simulink model "P1_secuencia"  (R2025a)
settings: Solver=ode23  StartTime=0.0  StopTime=T_SIM  MaxStep=0.01  RelTol=1e-3
PostLoadFcn:
  | run(fullfile(fileparts(get_param('P1_secuencia', 'FileName')), 'parametros_p1.m'));
InitFcn:
  | run(fullfile(fileparts(get_param('P1_secuencia', 'FileName')), 'parametros_p1.m'));
values from neighbouring files (symbols this model uses):
  CARRERA_13 = 100    [parametros_p1.m]
  CARRERA_45 = 50    [parametros_p1.m]
  DUR_START = 0.3    [parametros_p1.m]
  N_CICLOS = 3    [parametros_p1.m]
  P_CONM = 3    [parametros_p1.m]
  P_MIN_45 = 2    [parametros_p1.m]
  P_RED = 6    [parametros_p1.m]
  T_ESPERA = 1.0    (= 1)    [parametros_p1.m]
  T_NEUM = 5.0    (= 5)    [parametros_p1.m]
  T_START = 0.5    [parametros_p1.m]
  TAU_DESCARGA = 0.05    [parametros_p1.m]
  TAU_LINEA = 0.03    [parametros_p1.m]
  TAU_T1 = RETARDO_T1 / log(P_RED/(P_RED - P_CONM))    [parametros_p1.m]
  TAU_T2 = RETARDO_T2 / log(P_RED/(P_RED - P_CONM))    [parametros_p1.m]
  TOL_SENSOR = 1    [parametros_p1.m]
  V_EXT_13 = 100    [parametros_p1.m]
  V_EXT_45 = 100    [parametros_p1.m]
  V_RET_13 = 100    [parametros_p1.m]
  V_RET_45 = 125    [parametros_p1.m]
libraries: simulink x6
settings Model: Creator=Daan Maldonado  LastModifiedBy=Daan Maldonado

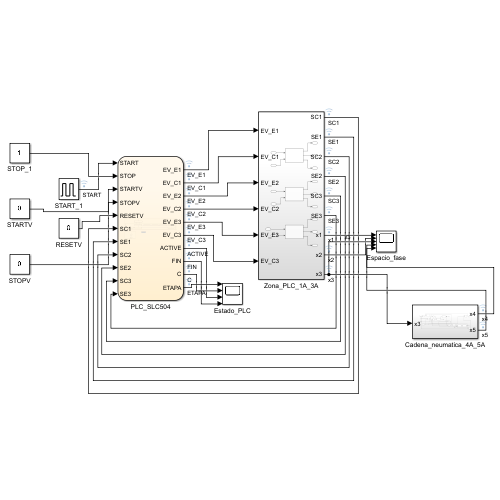
[thumbnail: Simulink's stored preview of the top-level diagram]
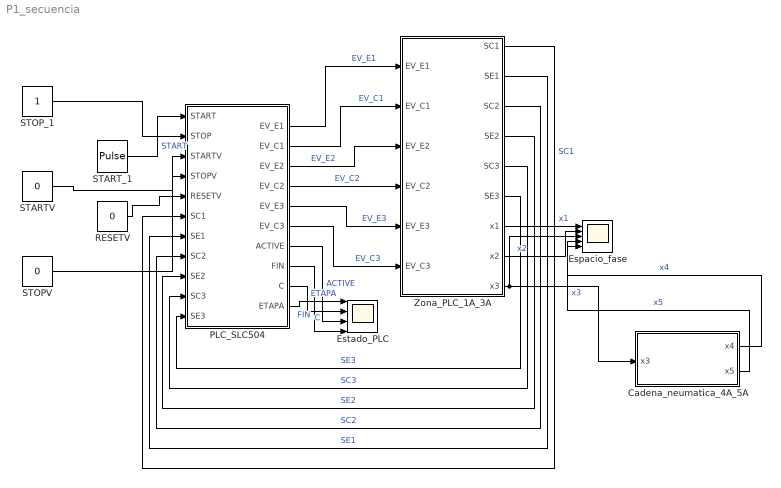
== system P1_secuencia ==
  Cadena_neumatica_4A_5A : Subsystem
  Espacio_fase : Scope  NumInputPorts=5
  Estado_PLC : Scope  NumInputPorts=4
  PLC_SLC504 : Stateflow chart  TreatAsAtomicUnit=on
  RESETV : Constant  Value=0
  STARTV : Constant  Value=0
  START_1 : DiscretePulseGenerator  PulseType=Time based  Period=1e4  PulseWidth=DUR_START/1e4*100  PhaseDelay=T_START
  STOPV : Constant  Value=0
  STOP_1 : Constant
  Zona_PLC_1A_3A : Subsystem
  wires:
  PLC_SLC504/8(FIN) -> Estado_PLC/4  "FIN"
  PLC_SLC504/7(ACTIVE) -> Estado_PLC/3  "ACTIVE"
  PLC_SLC504/9(C) -> Estado_PLC/2  "C"
  PLC_SLC504/10(ETAPA) -> Estado_PLC/1  "ETAPA"
  Cadena_neumatica_4A_5A/2(x5) -> Espacio_fase/5  "x5"
  Cadena_neumatica_4A_5A/1(x4) -> Espacio_fase/4  "x4"
  Zona_PLC_1A_3A/9(x3) -> Espacio_fase/3, Cadena_neumatica_4A_5A/1(x3)  "x3"
  Zona_PLC_1A_3A/8(x2) -> Espacio_fase/2  "x2"
  Zona_PLC_1A_3A/7(x1) -> Espacio_fase/1  "x1"
  Zona_PLC_1A_3A/6(SE3) -> PLC_SLC504/11(SE3)  "SE3"
  Zona_PLC_1A_3A/5(SC3) -> PLC_SLC504/10(SC3)  "SC3"
  Zona_PLC_1A_3A/4(SE2) -> PLC_SLC504/9(SE2)  "SE2"
  Zona_PLC_1A_3A/3(SC2) -> PLC_SLC504/8(SC2)  "SC2"
  Zona_PLC_1A_3A/2(SE1) -> PLC_SLC504/7(SE1)  "SE1"
  Zona_PLC_1A_3A/1(SC1) -> PLC_SLC504/6(SC1)  "SC1"
  PLC_SLC504/6(EV_C3) -> Zona_PLC_1A_3A/6(EV_C3)  "EV_C3"
  PLC_SLC504/5(EV_E3) -> Zona_PLC_1A_3A/5(EV_E3)  "EV_E3"
  PLC_SLC504/4(EV_C2) -> Zona_PLC_1A_3A/4(EV_C2)  "EV_C2"
  PLC_SLC504/3(EV_E2) -> Zona_PLC_1A_3A/3(EV_E2)  "EV_E2"
  PLC_SLC504/2(EV_C1) -> Zona_PLC_1A_3A/2(EV_C1)  "EV_C1"
  PLC_SLC504/1(EV_E1) -> Zona_PLC_1A_3A/1(EV_E1)  "EV_E1"
  RESETV/1 -> PLC_SLC504/5(RESETV)
  STOPV/1 -> PLC_SLC504/4(STOPV)
  STARTV/1 -> PLC_SLC504/3(STARTV)
  STOP_1/1 -> PLC_SLC504/2(STOP)
  START_1/1 -> PLC_SLC504/1(START)  "START"

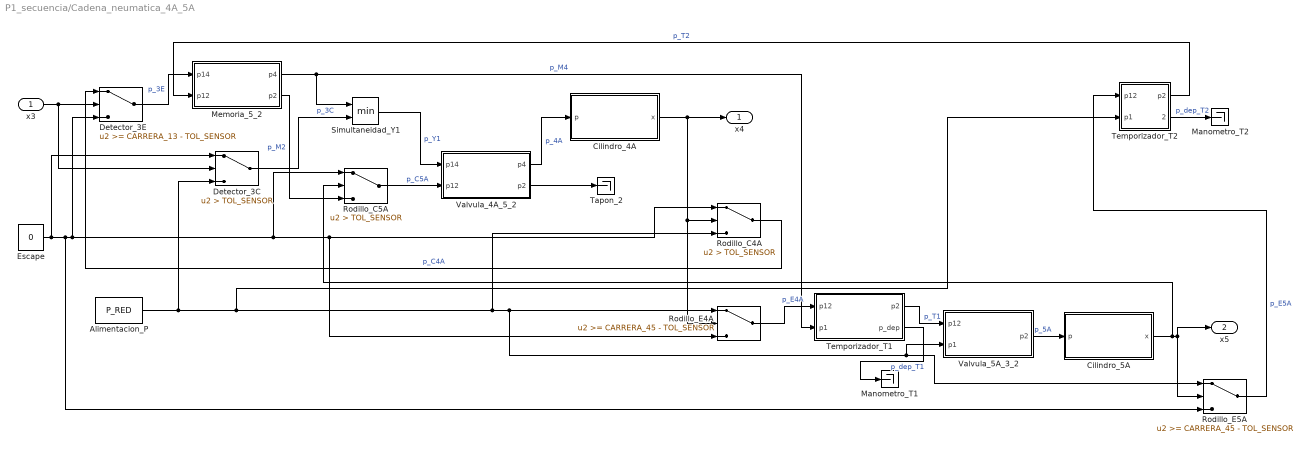
== system P1_secuencia/Cadena_neumatica_4A_5A ==
  x3 : Inport
  Alimentacion_P : Constant  Value=P_RED
  Cilindro_4A : Subsystem
  Cilindro_5A : Subsystem
  Detector_3C : Switch  Criteria=u2 > Threshold  Threshold=TOL_SENSOR  SaturateOnIntegerOverflow=off  InputSameDT=off
  Detector_3E : Switch  Threshold=CARRERA_13 - TOL_SENSOR  SaturateOnIntegerOverflow=off  InputSameDT=off
  Escape : Constant  Value=0
  Manometro_T1 : Terminator
  Manometro_T2 : Terminator
  Memoria_5_2 : Subsystem
  Rodillo_C4A : Switch  Criteria=u2 > Threshold  Threshold=TOL_SENSOR  SaturateOnIntegerOverflow=off  InputSameDT=off
  Rodillo_C5A : Switch  Criteria=u2 > Threshold  Threshold=TOL_SENSOR  SaturateOnIntegerOverflow=off  InputSameDT=off
  Rodillo_E4A : Switch  Threshold=CARRERA_45 - TOL_SENSOR  SaturateOnIntegerOverflow=off  InputSameDT=off
  Rodillo_E5A : Switch  Threshold=CARRERA_45 - TOL_SENSOR  SaturateOnIntegerOverflow=off  InputSameDT=off
  Simultaneidad_Y1 : MinMax  Inputs=2
  Tapon_2 : Terminator
  Temporizador_T1 : Subsystem
  Temporizador_T2 : Subsystem
  Valvula_4A_5_2 : Subsystem
  Valvula_5A_3_2 : Subsystem
  x4 : Outport
  x5 : Outport  Port=2
  wires:
  Memoria_5_2/2(p2) -> Rodillo_C5A/3  "p_M2"
  Cilindro_5A/1(x) -> x5/1, Rodillo_E5A/2, Rodillo_C5A/2
  Valvula_5A_3_2/1(p2) -> Cilindro_5A/1(p)  "p_5A"
  Temporizador_T1/1(p2) -> Valvula_5A_3_2/1(p12)  "p_T1"
  Rodillo_E4A/1 -> Temporizador_T1/1(p12)  "p_E4A"
  Cilindro_4A/1(x) -> Rodillo_E4A/2, Rodillo_C4A/2, x4/1
  Valvula_4A_5_2/2(p2) -> Tapon_2/1
  Valvula_4A_5_2/1(p4) -> Cilindro_4A/1(p)  "p_4A"
  Rodillo_C5A/1 -> Valvula_4A_5_2/2(p12)  "p_C5A"
  Simultaneidad_Y1/1 -> Valvula_4A_5_2/1(p14)  "p_Y1"
  Detector_3C/1 -> Simultaneidad_Y1/2  "p_3C"
  Memoria_5_2/1(p4) -> Simultaneidad_Y1/1, Temporizador_T1/2(p1)  "p_M4"
  Detector_3E/1 -> Memoria_5_2/1(p14)  "p_3E"
  Escape/1 -> Rodillo_E4A/3, Rodillo_C4A/1, Rodillo_C5A/1, Detector_3E/3, Rodillo_E5A/3, Detector_3C/1
  x3/1 -> Detector_3E/2, Detector_3C/2
  Rodillo_C4A/1 -> Detector_3E/1  "p_C4A"
  Temporizador_T2/2(p_dep) -> Manometro_T2/1  "p_dep_T2"
  Temporizador_T1/2(p_dep) -> Manometro_T1/1  "p_dep_T1"
  Alimentacion_P/1 -> Rodillo_E5A/1, Valvula_5A_3_2/2(p1), Rodillo_E4A/1, Rodillo_C4A/3, Temporizador_T2/2(p1), Detector_3C/3
  Temporizador_T2/1(p2) -> Memoria_5_2/2(p12)  "p_T2"
  Rodillo_E5A/1 -> Temporizador_T2/1(p12)  "p_E5A"

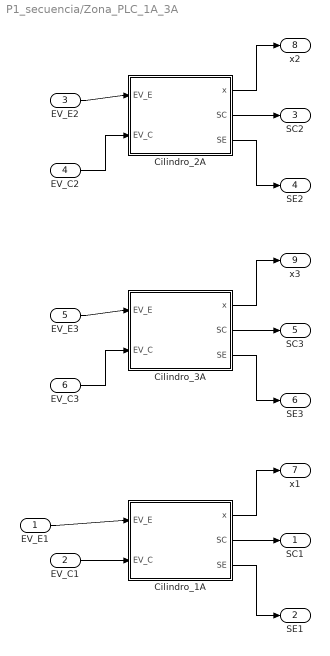
== system P1_secuencia/Zona_PLC_1A_3A ==
  EV_E1 : Inport
  EV_C1 : Inport  Port=2
  EV_E2 : Inport  Port=3
  EV_C2 : Inport  Port=4
  EV_E3 : Inport  Port=5
  EV_C3 : Inport  Port=6
  Cilindro_1A : Subsystem
  Cilindro_2A : Subsystem
  Cilindro_3A : Subsystem
  SC1 : Outport
  SE1 : Outport  Port=2
  SC2 : Outport  Port=3
  SE2 : Outport  Port=4
  SC3 : Outport  Port=5
  SE3 : Outport  Port=6
  x1 : Outport  Port=7
  x2 : Outport  Port=8
  x3 : Outport  Port=9
  wires:
  Cilindro_3A/3(SE) -> SE3/1
  Cilindro_3A/2(SC) -> SC3/1
  Cilindro_3A/1(x) -> x3/1
  Cilindro_2A/3(SE) -> SE2/1
  Cilindro_2A/2(SC) -> SC2/1
  Cilindro_2A/1(x) -> x2/1
  Cilindro_1A/3(SE) -> SE1/1
  Cilindro_1A/2(SC) -> SC1/1
  Cilindro_1A/1(x) -> x1/1
  EV_C3/1 -> Cilindro_3A/2(EV_C)
  EV_E3/1 -> Cilindro_3A/1(EV_E)
  EV_C2/1 -> Cilindro_2A/2(EV_C)
  EV_E2/1 -> Cilindro_2A/1(EV_E)
  EV_C1/1 -> Cilindro_1A/2(EV_C)
  EV_E1/1 -> Cilindro_1A/1(EV_E)

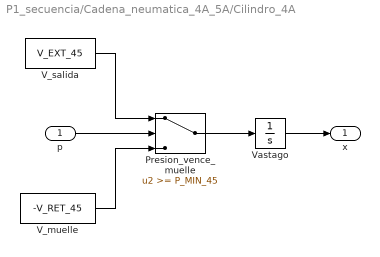
== system P1_secuencia/Cadena_neumatica_4A_5A/Cilindro_4A ==
  p : Inport
  Presion_vence_muelle : Switch  Threshold=P_MIN_45  SaturateOnIntegerOverflow=off  InputSameDT=off
  V_muelle : Constant  Value=-V_RET_45
  V_salida : Constant  Value=V_EXT_45
  Vastago : Integrator  LimitOutput=on  UpperSaturationLimit=CARRERA_45  LowerSaturationLimit=0
  x : Outport
  wires:
  Vastago/1 -> x/1
  Presion_vence_muelle/1 -> Vastago/1
  V_muelle/1 -> Presion_vence_muelle/3
  p/1 -> Presion_vence_muelle/2
  V_salida/1 -> Presion_vence_muelle/1

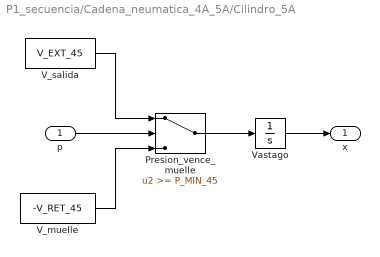
== system P1_secuencia/Cadena_neumatica_4A_5A/Cilindro_5A ==
  p : Inport
  Presion_vence_muelle : Switch  Threshold=P_MIN_45  SaturateOnIntegerOverflow=off  InputSameDT=off
  V_muelle : Constant  Value=-V_RET_45
  V_salida : Constant  Value=V_EXT_45
  Vastago : Integrator  LimitOutput=on  UpperSaturationLimit=CARRERA_45  LowerSaturationLimit=0
  x : Outport
  wires:
  Vastago/1 -> x/1
  Presion_vence_muelle/1 -> Vastago/1
  V_muelle/1 -> Presion_vence_muelle/3
  p/1 -> Presion_vence_muelle/2
  V_salida/1 -> Presion_vence_muelle/1

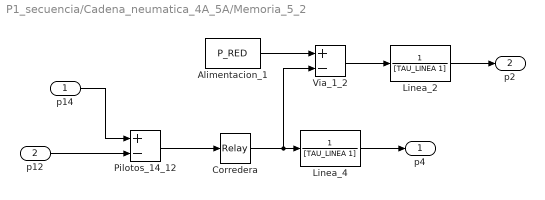
== system P1_secuencia/Cadena_neumatica_4A_5A/Memoria_5_2 ==
  p14 : Inport
  p12 : Inport  Port=2
  Alimentacion_1 : Constant  Value=P_RED
  Corredera : Relay  OnSwitchValue=P_CONM  OffSwitchValue=-P_CONM  OnOutputValue=P_RED
  Linea_2 : TransferFcn  Numerator=1  Denominator=[TAU_LINEA 1]
  Linea_4 : TransferFcn  Numerator=1  Denominator=[TAU_LINEA 1]
  Pilotos_14_12 : Sum  Inputs=+-
  Via_1_2 : Sum  Inputs=+-
  p4 : Outport
  p2 : Outport  Port=2
  wires:
  Linea_2/1 -> p2/1
  Via_1_2/1 -> Linea_2/1
  Alimentacion_1/1 -> Via_1_2/1
  Linea_4/1 -> p4/1
  Corredera/1 -> Linea_4/1, Via_1_2/2
  Pilotos_14_12/1 -> Corredera/1
  p12/1 -> Pilotos_14_12/2
  p14/1 -> Pilotos_14_12/1

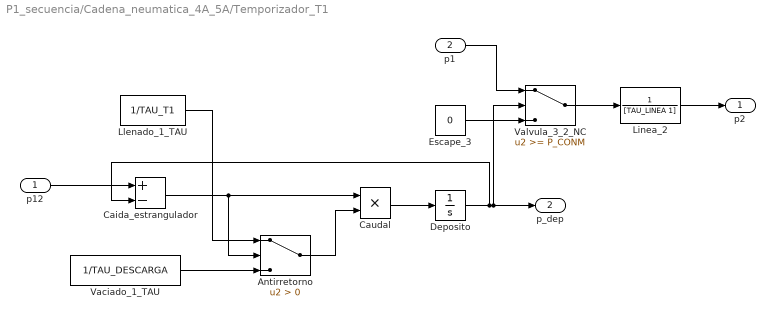
== system P1_secuencia/Cadena_neumatica_4A_5A/Temporizador_T1 ==
  p12 : Inport
  p1 : Inport  Port=2
  Antirretorno : Switch  Criteria=u2 > Threshold  SaturateOnIntegerOverflow=off  InputSameDT=off
  Caida_estrangulador : Sum  Inputs=+-
  Caudal : Product
  Deposito : Integrator
  Escape_3 : Constant  Value=0
  Linea_2 : TransferFcn  Numerator=1  Denominator=[TAU_LINEA 1]
  Llenado_1_TAU : Constant  Value=1/TAU_T1
  Vaciado_1_TAU : Constant  Value=1/TAU_DESCARGA
  Valvula_3_2_NC : Switch  Threshold=P_CONM  SaturateOnIntegerOverflow=off  InputSameDT=off
  p2 : Outport
  p_dep : Outport  Port=2
  wires:
  Linea_2/1 -> p2/1
  Valvula_3_2_NC/1 -> Linea_2/1
  Escape_3/1 -> Valvula_3_2_NC/3
  p1/1 -> Valvula_3_2_NC/1
  Caudal/1 -> Deposito/1
  Antirretorno/1 -> Caudal/2
  Vaciado_1_TAU/1 -> Antirretorno/3
  Caida_estrangulador/1 -> Caudal/1, Antirretorno/2
  Llenado_1_TAU/1 -> Antirretorno/1
  Deposito/1 -> Valvula_3_2_NC/2, p_dep/1, Caida_estrangulador/2
  p12/1 -> Caida_estrangulador/1

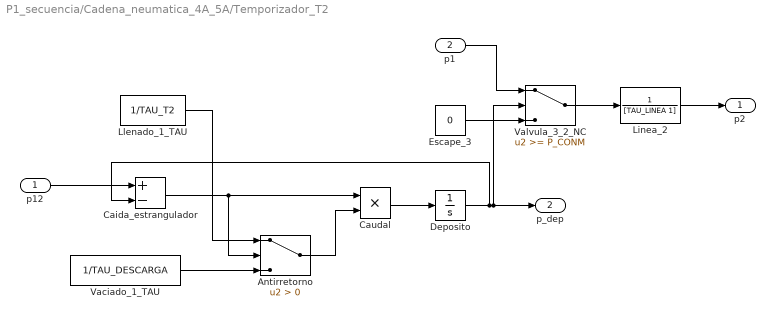
== system P1_secuencia/Cadena_neumatica_4A_5A/Temporizador_T2 ==
  p12 : Inport
  p1 : Inport  Port=2
  Antirretorno : Switch  Criteria=u2 > Threshold  SaturateOnIntegerOverflow=off  InputSameDT=off
  Caida_estrangulador : Sum  Inputs=+-
  Caudal : Product
  Deposito : Integrator
  Escape_3 : Constant  Value=0
  Linea_2 : TransferFcn  Numerator=1  Denominator=[TAU_LINEA 1]
  Llenado_1_TAU : Constant  Value=1/TAU_T2
  Vaciado_1_TAU : Constant  Value=1/TAU_DESCARGA
  Valvula_3_2_NC : Switch  Threshold=P_CONM  SaturateOnIntegerOverflow=off  InputSameDT=off
  p2 : Outport
  p_dep : Outport  Port=2
  wires:
  Linea_2/1 -> p2/1
  Valvula_3_2_NC/1 -> Linea_2/1
  Escape_3/1 -> Valvula_3_2_NC/3
  p1/1 -> Valvula_3_2_NC/1
  Caudal/1 -> Deposito/1
  Antirretorno/1 -> Caudal/2
  Vaciado_1_TAU/1 -> Antirretorno/3
  Caida_estrangulador/1 -> Caudal/1, Antirretorno/2
  Llenado_1_TAU/1 -> Antirretorno/1
  Deposito/1 -> Valvula_3_2_NC/2, p_dep/1, Caida_estrangulador/2
  p12/1 -> Caida_estrangulador/1

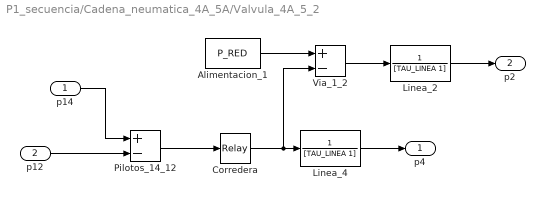
== system P1_secuencia/Cadena_neumatica_4A_5A/Valvula_4A_5_2 ==
  p14 : Inport
  p12 : Inport  Port=2
  Alimentacion_1 : Constant  Value=P_RED
  Corredera : Relay  OnSwitchValue=P_CONM  OffSwitchValue=-P_CONM  OnOutputValue=P_RED
  Linea_2 : TransferFcn  Numerator=1  Denominator=[TAU_LINEA 1]
  Linea_4 : TransferFcn  Numerator=1  Denominator=[TAU_LINEA 1]
  Pilotos_14_12 : Sum  Inputs=+-
  Via_1_2 : Sum  Inputs=+-
  p4 : Outport
  p2 : Outport  Port=2
  wires:
  Linea_2/1 -> p2/1
  Via_1_2/1 -> Linea_2/1
  Alimentacion_1/1 -> Via_1_2/1
  Linea_4/1 -> p4/1
  Corredera/1 -> Linea_4/1, Via_1_2/2
  Pilotos_14_12/1 -> Corredera/1
  p12/1 -> Pilotos_14_12/2
  p14/1 -> Pilotos_14_12/1

== system P1_secuencia/Cadena_neumatica_4A_5A/Valvula_5A_3_2 ==
  p12 : Inport
  p1 : Inport  Port=2
  Corredera_muelle : Switch  Threshold=P_CONM  SaturateOnIntegerOverflow=off  InputSameDT=off
  Escape_3 : Constant  Value=0
  Linea_2 : TransferFcn  Numerator=1  Denominator=[TAU_LINEA 1]
  p2 : Outport
  wires:
  Linea_2/1 -> p2/1
  Corredera_muelle/1 -> Linea_2/1
  Escape_3/1 -> Corredera_muelle/3
  p12/1 -> Corredera_muelle/2
  p1/1 -> Corredera_muelle/1

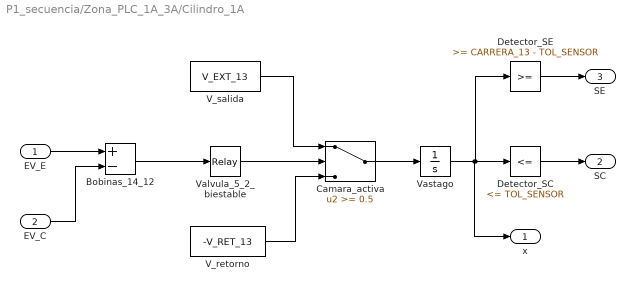
== system P1_secuencia/Zona_PLC_1A_3A/Cilindro_1A ==
  EV_E : Inport
  EV_C : Inport  Port=2
  Bobinas_14_12 : Sum  Inputs=+-
  Camara_activa : Switch  Threshold=0.5  SaturateOnIntegerOverflow=off  InputSameDT=off
  Detector_SC : simulink/Logic and Bit Operations/Compare To Constant  relop=<=  const=TOL_SENSOR  OutDataTypeStr=boolean
  Detector_SE : simulink/Logic and Bit Operations/Compare To Constant  relop=>=  const=CARRERA_13 - TOL_SENSOR  OutDataTypeStr=boolean
  V_retorno : Constant  Value=-V_RET_13
  V_salida : Constant  Value=V_EXT_13
  Valvula_5_2_biestable : Relay  OnSwitchValue=0.5  OffSwitchValue=-0.5
  Vastago : Integrator  LimitOutput=on  UpperSaturationLimit=CARRERA_13  LowerSaturationLimit=0
  x : Outport
  SC : Outport  Port=2
  SE : Outport  Port=3
  wires:
  Detector_SE/1 -> SE/1
  Detector_SC/1 -> SC/1
  Vastago/1 -> Detector_SC/1, Detector_SE/1, x/1
  Camara_activa/1 -> Vastago/1
  V_retorno/1 -> Camara_activa/3
  Valvula_5_2_biestable/1 -> Camara_activa/2
  V_salida/1 -> Camara_activa/1
  Bobinas_14_12/1 -> Valvula_5_2_biestable/1
  EV_C/1 -> Bobinas_14_12/2
  EV_E/1 -> Bobinas_14_12/1

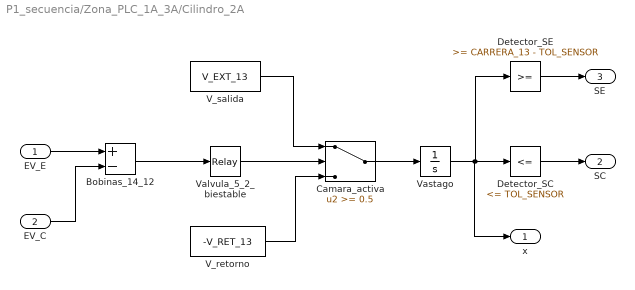
== system P1_secuencia/Zona_PLC_1A_3A/Cilindro_2A ==
  EV_E : Inport
  EV_C : Inport  Port=2
  Bobinas_14_12 : Sum  Inputs=+-
  Camara_activa : Switch  Threshold=0.5  SaturateOnIntegerOverflow=off  InputSameDT=off
  Detector_SC : simulink/Logic and Bit Operations/Compare To Constant  relop=<=  const=TOL_SENSOR  OutDataTypeStr=boolean
  Detector_SE : simulink/Logic and Bit Operations/Compare To Constant  relop=>=  const=CARRERA_13 - TOL_SENSOR  OutDataTypeStr=boolean
  V_retorno : Constant  Value=-V_RET_13
  V_salida : Constant  Value=V_EXT_13
  Valvula_5_2_biestable : Relay  OnSwitchValue=0.5  OffSwitchValue=-0.5
  Vastago : Integrator  LimitOutput=on  UpperSaturationLimit=CARRERA_13  LowerSaturationLimit=0
  x : Outport
  SC : Outport  Port=2
  SE : Outport  Port=3
  wires:
  Detector_SE/1 -> SE/1
  Detector_SC/1 -> SC/1
  Vastago/1 -> Detector_SC/1, Detector_SE/1, x/1
  Camara_activa/1 -> Vastago/1
  V_retorno/1 -> Camara_activa/3
  Valvula_5_2_biestable/1 -> Camara_activa/2
  V_salida/1 -> Camara_activa/1
  Bobinas_14_12/1 -> Valvula_5_2_biestable/1
  EV_C/1 -> Bobinas_14_12/2
  EV_E/1 -> Bobinas_14_12/1

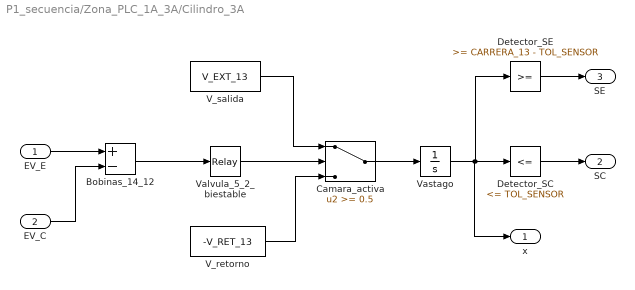
== system P1_secuencia/Zona_PLC_1A_3A/Cilindro_3A ==
  EV_E : Inport
  EV_C : Inport  Port=2
  Bobinas_14_12 : Sum  Inputs=+-
  Camara_activa : Switch  Threshold=0.5  SaturateOnIntegerOverflow=off  InputSameDT=off
  Detector_SC : simulink/Logic and Bit Operations/Compare To Constant  relop=<=  const=TOL_SENSOR  OutDataTypeStr=boolean
  Detector_SE : simulink/Logic and Bit Operations/Compare To Constant  relop=>=  const=CARRERA_13 - TOL_SENSOR  OutDataTypeStr=boolean
  V_retorno : Constant  Value=-V_RET_13
  V_salida : Constant  Value=V_EXT_13
  Valvula_5_2_biestable : Relay  OnSwitchValue=0.5  OffSwitchValue=-0.5
  Vastago : Integrator  LimitOutput=on  UpperSaturationLimit=CARRERA_13  LowerSaturationLimit=0
  x : Outport
  SC : Outport  Port=2
  SE : Outport  Port=3
  wires:
  Detector_SE/1 -> SE/1
  Detector_SC/1 -> SC/1
  Vastago/1 -> Detector_SC/1, Detector_SE/1, x/1
  Camara_activa/1 -> Vastago/1
  V_retorno/1 -> Camara_activa/3
  Valvula_5_2_biestable/1 -> Camara_activa/2
  V_salida/1 -> Camara_activa/1
  Bobinas_14_12/1 -> Valvula_5_2_biestable/1
  EV_C/1 -> Bobinas_14_12/2
  EV_E/1 -> Bobinas_14_12/1

== stateflow chart P1_secuencia/PLC_SLC504 ==
  settings: updateMethod=DISCRETE  sampleTime=Ts_PLC
  state GP [parallel]
    settings: executionOrder=2
    state X0
      en, du: ETAPA = 0; salidas(0, SE1, 0, SE2, 0, SE3);
    state CICLO
      state X1
        en, du: ETAPA = 1; salidas(1, 0, 0, 0, 0, 0);
      state X2
        en, du: ETAPA = 2; DN = elapsed(sec) >= T_ESPERA;
        salidas(~DN, DN, 0, 0, 0, 0);
      state X3
        en, du: ETAPA = 3; DN = elapsed(sec) >= T_ESPERA;
        salidas(0, ~DN, DN, 0, 0, 0);
      state X4
        en, du: ETAPA = 4; DN = elapsed(sec) >= T_ESPERA;
        salidas(0, 0, ~DN, DN, 0, 0);
      state X5
        en, du: ETAPA = 5; DN = elapsed(sec) >= T_ESPERA;
        salidas(0, 0, 0, ~DN, DN, 0);
      state X7
        en: C = C + 1; ETAPA = 7; salidas(0, 0, 0, 0, 0, 1);
        du: DN = elapsed(sec) >= T_NEUM;
        salidas(0, DN && SE1, 0, DN && SE2, 0, ~DN || SE3);
      state X8
        en: ETAPA = 8; FIN = 1; salidas(0, 0, 0, 0, 0, 0);
        ex: FIN = 0;
      state X6
        en, du: ETAPA = 6; DN = elapsed(sec) >= T_ESPERA;
        salidas(0, 0, 0, 0, ~DN, DN);
      X1 -> X2 : [ACTIVE && SE1]
      X2 -> X3 : [after(T_ESPERA, sec) && ACTIVE && SC1]
      X3 -> X4 : [after(T_ESPERA, sec) && ACTIVE && SE2]
      X4 -> X5 : [after(T_ESPERA, sec) && ACTIVE && SC2]
      X5 -> X6 : [after(T_ESPERA, sec) && ACTIVE && SE3]
      X7 -> X1 [order 1] : [after(T_NEUM, sec) && ACTIVE && SC3 && C < N_CICLOS]
      X7 -> X8 [order 2] : [after(T_NEUM, sec) && ACTIVE && C >= N_CICLOS]
      X6 -> X7 : [after(T_ESPERA, sec) && ACTIVE && SC3]
    (default) -> X0
    CICLO -> X0 : [FIN || (START && ~STOP) || RESETV]{C = 0;}
    X0 -> X1 : [ACTIVE && SC1 && SC2 && SC3 && (START || STARTV)]
  state GM [parallel]
    settings: executionOrder=1
    state X10
      en: ACTIVE = 0;
    state X11
      en: ACTIVE = 1;
    (default) -> X10
    X11 -> X10 : [~STOP || STOPV || FIN]
    X10 -> X11 : [(START || STARTV) && STOP && ~STOPV && ~FIN]
  data: e1 function_input; c1 function_input; e2 function_input; c2 function_input; e3 function_input; c3 function_input; START input double; STOP input double; STARTV input double; STOPV input double; RESETV input double; SC1 input boolean; SE1 input boolean; SC2 input boolean; SE2 input boolean; SC3 input boolean; SE3 input boolean; T_ESPERA parameter double; T_NEUM parameter double; N_CICLOS parameter double; EV_E1 output double =0; EV_C1 output double =0; EV_E2 output double =0; EV_C2 output double =0; EV_E3 output double =0; EV_C3 output double =0; ACTIVE output double =0; FIN output double =0; C output double =0; ETAPA output double =0; DN local boolean =false
  function salidas(e1, c1, e2, c2, e3, c3):
    | function salidas(e1, c1, e2, c2, e3, c3)
    | % Escribe las bobinas O:2/0..5 (EV_E1, EV_C1, EV_E2, EV_C2, EV_E3, EV_C3).
    | EV_E1 = double(e1);
    | EV_C1 = double(c1);
    | EV_E2 = double(e2);
    | EV_C2 = double(c2);
    | EV_E3 = double(e3);
    | EV_C3 = double(c3);
    | end
